simulink model "new_MASH"  (R2022b)
settings: Solver=VariableStepAuto  StartTime=0.0  StopTime=0.01  RelTol=1e-3
undefined symbols (not defined in the file or in its folder): dspblkCoreblockFVToolHelper, gcbh
libraries: dspsrcs4 x1
settings Model: Creator=khaled  LastModifiedBy=khaled
settings OptimizationCC: ReuseModelBlockBuffer=on
settings RTWCC: GPUComputeCapability=5.0

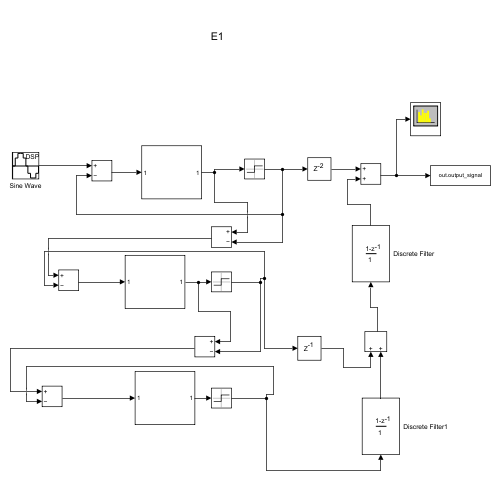
[thumbnail: Simulink's stored preview of the top-level diagram]
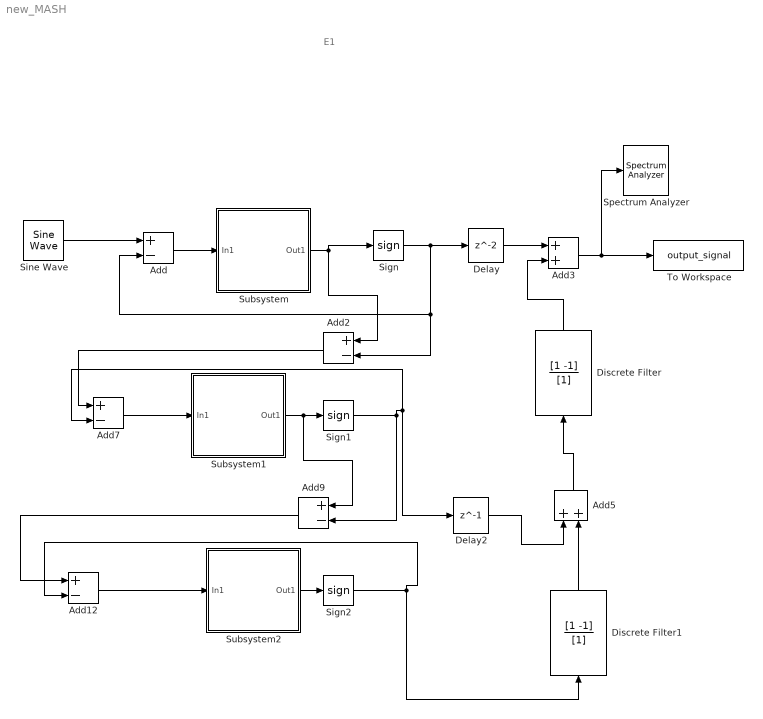
== system new_MASH ==
  note: E1
  Add{,2,7,9,12} (5 alike) : Sum  Inputs=+-
  Add3 : Sum
  Add5 : Sum
  Delay : Delay
  Delay2 : Delay  DelayLength=1  InputProcessing=Columns as channels (frame based)
  Discrete Filter : DiscreteFilter  LoadFcn=dspblkCoreblockFVToolHelper(gcbh,'load');  Numerator=[1 -1]  Denominator=[1]  InputProcessing=Columns as channels (frame based)  FilterStructure=Direct form II transposed  a0EqualsOne=on
      settings: CopyFcn=dspblkCoreblockFVToolHelper(gcbh,'copy');  DeleteFcn=dspblkCoreblockFVToolHelper(gcbh,'close');  ModelCloseFcn=dspblkCoreblockFVToolHelper(gcbh,'close');  PreSaveFcn=dspblkCoreblockFVToolHelper(gcbh,'presave');  PostSaveFcn=dspblkCoreblockFVToolHelper(gcbh,'postsave');  CloseFcn=dspblkCoreblockFVToolHelper(gcbh,'close');
  Discrete Filter1 : DiscreteFilter  LoadFcn=dspblkCoreblockFVToolHelper(gcbh,'load');  Numerator=[1 -1]  Denominator=[1]  InputProcessing=Columns as channels (frame based)  FilterStructure=Direct form II transposed  a0EqualsOne=on
      settings: CopyFcn=dspblkCoreblockFVToolHelper(gcbh,'copy');  DeleteFcn=dspblkCoreblockFVToolHelper(gcbh,'close');  ModelCloseFcn=dspblkCoreblockFVToolHelper(gcbh,'close');  PreSaveFcn=dspblkCoreblockFVToolHelper(gcbh,'presave');  PostSaveFcn=dspblkCoreblockFVToolHelper(gcbh,'postsave');  CloseFcn=dspblkCoreblockFVToolHelper(gcbh,'close');
  Sign : Signum
  Sign1 : Signum
  Sign2 : Signum
  Sine Wave : dspsrcs4/Sine Wave  Amplitude=1  Frequency=100e3  Phase=0  SampleMode=Discrete  OutComplex=Real  CompMethod=Trigonometric fcn  TableSize=Speed  SampleTime=1e-8  SamplesPerFrame=1  ResetState=Restart at time zero  OutputFrames=off  dataType=double  wordLen=16  udDataType=sfix(16)  fracBitsMode=Best precision  numFracBits=15  OutDataTypeStr=double  LastOutDataTypeStr=double
  Spectrum Analyzer : SpectrumAnalyzer  DefaultConfigurationName=spbscopes.SpectrumAnalyzerBlockCfg
  Subsystem : Subsystem
  Subsystem1 : Subsystem
  Subsystem2 : Subsystem
  To Workspace : ToWorkspace  VariableName=output_signal  SaveFormat=Timeseries  SampleTime=-1
  wires:
  Sine Wave/1 -> Add/1
  Sign/1 -> Add2/2, Add/2, Delay/1
  Delay/1 -> Add3/1
  Add3/1 -> To Workspace/1, Spectrum Analyzer/1
  Delay2/1 -> Add5/1
  Add2/1 -> Add7/1
  Add/1 -> Subsystem/1(In1)
  Subsystem/1(Out1) -> Add2/1, Sign/1
  Subsystem1/1(Out1) -> Sign1/1, Add9/1
  Add7/1 -> Subsystem1/1(In1)
  Sign1/1 -> Add7/2, Delay2/1, Add9/2
  Subsystem2/1(Out1) -> Sign2/1
  Add12/1 -> Subsystem2/1(In1)
  Sign2/1 -> Add12/2, Discrete Filter1/1
  Add9/1 -> Add12/1
  Discrete Filter/1 -> Add3/2
  Add5/1 -> Discrete Filter/1
  Discrete Filter1/1 -> Add5/2

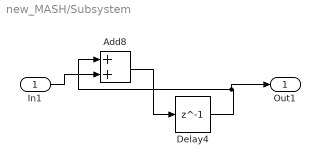
== system new_MASH/Subsystem ==
  In1 : Inport
  Add8 : Sum
  Delay4 : Delay  DelayLength=1  InputProcessing=Columns as channels (frame based)
  Out1 : Outport
  wires:
  Delay4/1 -> Out1/1, Add8/1
  Add8/1 -> Delay4/1
  In1/1 -> Add8/2

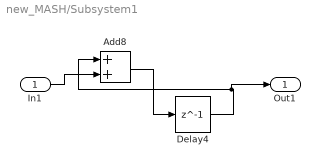
== system new_MASH/Subsystem1 ==
  In1 : Inport
  Add8 : Sum
  Delay4 : Delay  DelayLength=1  InputProcessing=Columns as channels (frame based)
  Out1 : Outport
  wires:
  Delay4/1 -> Out1/1, Add8/1
  Add8/1 -> Delay4/1
  In1/1 -> Add8/2

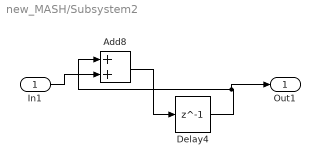
== system new_MASH/Subsystem2 ==
  In1 : Inport
  Add8 : Sum
  Delay4 : Delay  DelayLength=1  InputProcessing=Columns as channels (frame based)
  Out1 : Outport
  wires:
  Delay4/1 -> Out1/1, Add8/1
  Add8/1 -> Delay4/1
  In1/1 -> Add8/2
